simulink model "gtm_design"  (R2021b)
settings: Solver=VariableStepAuto  StartTime=0.0  StopTime=30  MinStep=0.0049  RelTol=1e-3
StopFcn:
  | MWSout=grabmws(bdroot);
  | MWSout.lastrun=datestr(now);
values from neighbouring files (symbols this model uses):
  g = 32.17405    [SingleDOF.m]    (also in layer1atm.m; mainSimple.m = 32.174; simio.m = [dx(Index.EOM(1:6)); delta(:)-f; -delta(:)-f ])
  GuidanceMode = 1    [mainSimple.m]    (also in setup.m)
  knots2fps = 1/fps2knots    (= 1.687800745)    [main.m]    (also in mainSimple.m = 1.68781)
  s = tf('s')    [SingleDOF.m]    (also in main.m; mainSimple.m; newmain.m)
undefined symbols (not defined in the file or in its folder): Aero, aftfuel, aftfuel_pos, AILL, AILLC, AILR, AILRC, alpha_deg, altitude_ft, Ax_g, Ay_g, Az_g, b, beta_deg, bias, BRAKEC, Cbar, cg_pos0, cg_shift_gear, DamageCase, DamageModels, DamageOnsetTime, Earth, ELLIB, ELLIBC, ELLOB, ELLOBC, ELRIB, ELRIBC, ELROB, ELROBC, engl_ang, engl_pos, engr_ang, engr_pos, FLAPLC, FLAPLIB, FLAPLOB, FLAPRC, FLAPRIB, FLAPROB, FuelUsed_Init, fwdfuel, fwdfuel_pos, GEAR, GEARC, Inertia0, Inertia_shift_gear, Ixx_model, Iyy_model, Izz_model, KTAS, LandingGear, LengON, LinearizeModeOn, m, MORPHLC, MORPHRC, NAV_altitude_m, NAV_latitude_deg ... (+51)
libraries: simulink_extras x39, simulink_need_slupdate x30, LPVBlockLibrary x9, aerolibconvert2 x7, simulink x3, aerolibtransform2 x3, UserContent_lib x2, uavalgslib x2, robotcorelib x1, uavutilslib x1
(part 1 of 7)
settings Model: VariantFading=off  LastModifiedBy=Jihoon Lee
settings DataIOCC: ReturnWorkspaceOutputs=off
settings OptimizationCC: BlockReduction=off  BooleanDataType=off
settings DebuggingCC: SaveWithParameterizedLinksMsg=none  UnderspecifiedInitializationDetection=Classic  MergeDetectMultiDrivingBlocksExec=none  SignalResolutionControl=TryResolveAllWithWarning
settings HardwareCC: TargetUnknown=on
settings ModelReferenceCC: PropagateSignalLabelsOutOfModel=off

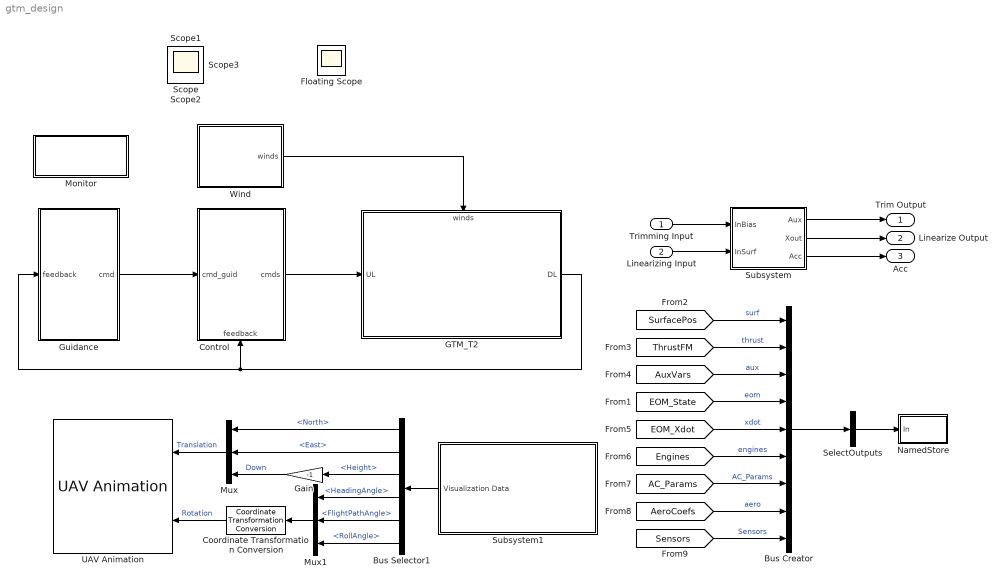
== system gtm_design ==
  Trimming Input : Inport  OutDataTypeStr=double  PortDimensions=4
  Linearizing Input : Inport  Port=2  OutDataTypeStr=double  PortDimensions=19
  Bus Creator : BusCreator  Inputs=9
  Bus Selector1 : BusSelector  OutputSignals=North,East,Height,HeadingAngle,FlightPathAngle,RollAngle
  Control : Subsystem
      settings: PortSchema="{\"entries\":[{\"content\":{\"sides\":[{\"content\":{\"connectorIds\":[\"In1\"]},\"type\":\"ConnectorPlacement.EquallySpacedRectSide\",\"uuid\":\"876f9d1c-31d1-4d48-8cbb-f6088518770e\"},{\"content\":{\"connectorIds\":[\"Out1\"],\"side\":\"RIGHT\"},\"type\":\"ConnectorPlacement.EquallySpacedRectSide\",\"uuid\":\"0e4266e3-a031-465f-8381-066e8420e2a4\"},{\"content\":{\"connectorIds\":[],\"side\":\"TOP\"},\"type\":\"ConnectorPlacement.EquallySpacedRectSide\",\"uuid\":\"3957ab9c-ff96-432b-bd6f-14b7cf2f8092\"},{\"content\":{\"connectorIds\":[\"In2\"],\"side\":\"BOTTOM\"},\"type\":\"ConnectorPlacement.EquallySpacedRectSide\",\"uuid\":\"1e447cfa-7c82-4ae0-9a3c-28fe1a02d81e\"}]},\"type\":\"ConnectorPlacement.EquallySpacedConnector\",\"uuid\":\"5c345d19-69a3-46c5-b9cf-f35f763eae5c\"}],\"packageUris\":[\"http://schema.mathworks.com/mf0/Connector/R2020b\"],\"version\":\"1.0\"}"
  Coordinate Transformation Conversion : robotcorelib/Coordinate Transformation Conversion  InputRepresentation=Euler Angles  InputEulerSequence=ZYX  ShowTrVecInputPort=on  OutputRepresentation=Quaternion  OutputEulerSequence=ZYX  ShowTrVecOutputPort=on  SimulateUsing=Code generation
      settings: SourceProductBaseCode=NV,RO,RR,UV
  GTM_T2 : Subsystem  Tag=From trunk/GTMsim/gtm_model.mdl revision 162
      settings: PortSchema="{\"entries\":[{\"content\":{\"sides\":[{\"content\":{\"connectorIds\":[\"In1\"]},\"type\":\"ConnectorPlacement.EquallySpacedRectSide\",\"uuid\":\"38bba5f1-4a0f-4ecd-874d-3a7e9850121a\"},{\"content\":{\"connectorIds\":[\"Out1\"],\"side\":\"RIGHT\"},\"type\":\"ConnectorPlacement.EquallySpacedRectSide\",\"uuid\":\"3320f707-8849-454c-b6a8-a1a5600dce96\"},{\"content\":{\"connectorIds\":[\"In2\"],\"side\":\"TOP\"},\"type\":\"ConnectorPlacement.EquallySpacedRectSide\",\"uuid\":\"e35b4c5d-b5fc-496b-a614-8f47a0366b54\"}]},\"type\":\"ConnectorPlacement.EquallySpacedConnector\",\"uuid\":\"76f2ccd8-2b0a-475c-a3e4-032abf049833\"}],\"packageUris\":[\"http://schema.mathworks.com/mf0/Connector/R2020b\"],\"version\":\"1.0\"}"
      mask Display: image(imread('GTMtiny.png'))
  Gain : Gain  Gain=-1
  Guidance : Subsystem
  Monitor : Subsystem
  Mux : Mux  Inputs=3
  Mux1 : Mux  Inputs=3
  NamedStore : Subsystem  StopFcn=|  mask{enable_logging=on, do_stopfcn_callback=on}
      | % if strmatch(get_param(gcb,'do_stopfcn_callback'),...
      | % 'on','exact')                                       
      | %    if exist('logsout','var')                        
      | %        sout = CreateSimOut(logsout);                
      | %    else                                             
      | %         %disp('No Log Data Variable')               
      | %     end                                             
      | % clear logsout                                       
      | % end
      mask prompts: enable_logging "Enable Data Logging"; do_stopfcn_callback "Post-process logsout"
      mask help: Produces signal log of input data. If post processing is selected the logsout object is converted into a data structure (sout) with fields named after the bus signals. In this case a common time base is recommended.
      mask init:
      | H=get_param([gcb,'/In'],'PortHandles');
      | if (enable_logging)
      |     set(H.Outport(1),'DataLogging','on')
      | else
      |     set(H.Outport(1),'DataLogging','off')
      |     
      | end
  SelectOutputs : BusSelector  OutputSignals=surf,thrust,aux,eom,xdot,engines,AC_Params,aero,Sensors  OutputAsBus=on
  Subsystem : Subsystem
  Subsystem1 : Subsystem
  UAV Animation : uavutilslib/UAV Animation  UAVType=FixedWing  UAVSize=50  InertialZDirection=Down  SampleTime=1
      settings: SourceProductBaseCode=UV
  Wind : Subsystem
  Trim Output : Outport  OutDataTypeStr=double  PortDimensions=6
  Linearize Output : Outport  Port=2  OutDataTypeStr=double  PortDimensions=12
  Acc : Outport  Port=3  OutDataTypeStr=double  PortDimensions=3
  Floating Scope : Scope
  Scope{,1..3} (4 alike) : Scope
  wires:
  Linearizing Input/1 -> Subsystem/2(InSurf)
  Subsystem/1(Aux) -> Trim Output/1
  Subsystem/2(Xout) -> Linearize Output/1
  Trimming Input/1 -> Subsystem/1(InBias)
  Control/1(cmds) -> GTM_T2/1(UL)
  Subsystem/3(Acc) -> Acc/1
  Bus Selector1/6 -> Mux1/3  "<RollAngle>"
  Mux/1 -> UAV Animation/1  "Translation"
  Bus Selector1/2 -> Mux/2  "<East>"
  Mux1/1 -> Coordinate Transformation Conversion/1
  Bus Selector1/1 -> Mux/1  "<North>"
  Bus Selector1/4 -> Mux1/1  "<HeadingAngle>"
  Coordinate Transformation Conversion/1 -> UAV Animation/2  "Rotation"
  Bus Selector1/3 -> Gain/1  "<Height>"
  Bus Selector1/5 -> Mux1/2  "<FlightPathAngle>"
  Gain/1 -> Mux/3  "Down"
  GTM_T2/1(DL) -> Guidance/1(feedback), Control/2(feedback)
  Guidance/1(cmd) -> Control/1(cmd_guid)
  Subsystem1/1(Visualization Data) -> Bus Selector1/1
  SelectOutputs/1 -> NamedStore/1(In)
  [AuxVars] -> Bus Creator/3  "aux"
  [ThrustFM] -> Bus Creator/2  "thrust"
  Bus Creator/1 -> SelectOutputs/1
  [SurfacePos] -> Bus Creator/1  "surf"
  [Sensors] -> Bus Creator/9  "Sensors"
  [Engines] -> Bus Creator/6  "engines"
  [EOM_Xdot] -> Bus Creator/5  "xdot"
  [AeroCoefs] -> Bus Creator/8  "aero"
  [AC_Params] -> Bus Creator/7  "AC_Params"
  [EOM_State] -> Bus Creator/4  "eom"
  Wind/1(winds) -> GTM_T2/2(winds)

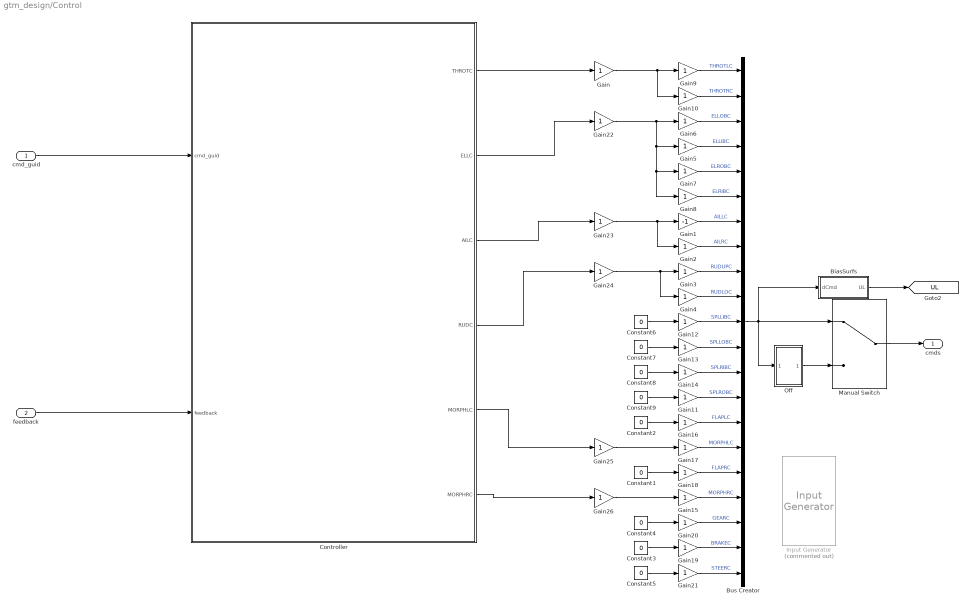
== system gtm_design/Control ==
  cmd_guid : Inport
  feedback : Inport  Port=2
  BiasSurfs : Subsystem
  Bus Creator : BusCreator  Inputs=21
  Constant{1..9} (9 alike) : Constant  Value=0
  Controller : Subsystem
  Gain{,22..26} (6 alike) : Gain
  Gain1 : Gain  Gain=-1  SaturateOnIntegerOverflow=on  OutDataTypeStr=Inherit: Same as input  ParamDataTypeStr=Inherit: Same as input
  Gain{2..21} (20 alike) : Gain  SaturateOnIntegerOverflow=on  OutDataTypeStr=Inherit: Same as input  ParamDataTypeStr=Inherit: Same as input
  Input Generator : UserContent_lib/Input Generator  Commented=on  SystemSampleTime=-1  VariantActivationTime=update diagram  Latency=0  AutoFrameSizeCalculation=off
      link override Doublet Generator: timeon=[2 12 7]  pulsewidth=[0.5 0.5 0.5]  amplitude=[0 0 0]
  Manual Switch : ManualSwitch
  Off : Subsystem
  cmds : Outport
  tag scope: UL=global
  wires:
  Gain9/1 -> Bus Creator/1  "THROTLC"
  Gain17/1 -> Bus Creator/16  "MORPHLC"
  Gain5/1 -> Bus Creator/4  "ELLIBC"
  Gain20/1 -> Bus Creator/19  "GEARC"
  Gain11/1 -> Bus Creator/14  "SPLROBC"
  Gain8/1 -> Bus Creator/6  "ELRIBC"
  Gain13/1 -> Bus Creator/12  "SPLLOBC"
  Gain1/1 -> Bus Creator/7  "AILLC"
  Gain7/1 -> Bus Creator/5  "ELROBC"
  Gain15/1 -> Bus Creator/18  "MORPHRC"
  Constant4/1 -> Gain20/1
  Gain2/1 -> Bus Creator/8  "AILRC"
  Gain3/1 -> Bus Creator/9  "RUDUPC"
  Gain21/1 -> Bus Creator/21  "STEERC"
  Gain14/1 -> Bus Creator/13  "SPLRIBC"
  Constant3/1 -> Gain19/1
  Gain6/1 -> Bus Creator/3  "ELLOBC"
  Gain10/1 -> Bus Creator/2  "THROTRC"
  Gain19/1 -> Bus Creator/20  "BRAKEC"
  Gain18/1 -> Bus Creator/17  "FLAPRC"
  Gain4/1 -> Bus Creator/10  "RUDLOC"
  Bus Creator/1 -> Off/1(In1), BiasSurfs/1(dCmd), Manual Switch/1
  Gain12/1 -> Bus Creator/11  "SPLLIBC"
  Gain16/1 -> Bus Creator/15  "FLAPLC"
  Constant2/1 -> Gain16/1
  Controller/3(AILC) -> Gain23/1
  Controller/2(ELLC) -> Gain22/1
  Controller/4(RUDC) -> Gain24/1
  Controller/1(THROTC) -> Gain/1
  cmd_guid/1 -> Controller/1(cmd_guid)
  feedback/1 -> Controller/2(feedback)
  Constant1/1 -> Gain18/1
  Constant5/1 -> Gain21/1
  Constant6/1 -> Gain12/1
  Constant7/1 -> Gain13/1
  Constant8/1 -> Gain14/1
  Constant9/1 -> Gain11/1
  Controller/5(MORPHLC) -> Gain25/1
  Controller/6(MORPHRC) -> Gain26/1
  Gain/1 -> Gain10/1, Gain9/1
  Gain22/1 -> Gain8/1, Gain7/1, Gain5/1, Gain6/1
  Gain23/1 -> Gain2/1, Gain1/1
  Gain24/1 -> Gain4/1, Gain3/1
  Gain25/1 -> Gain17/1
  Gain26/1 -> Gain15/1
  Manual Switch/1 -> cmds/1
  Off/1(Out1) -> Manual Switch/2
  BiasSurfs/1(UL) -> [UL]

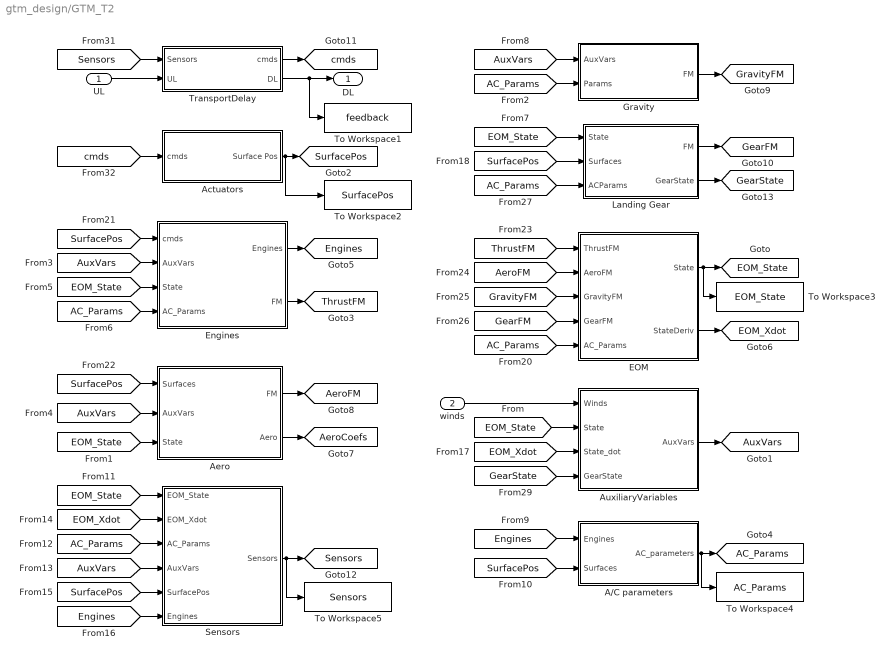
== system gtm_design/GTM_T2 ==
  UL : Inport
  winds : Inport  Port=2  PortDimensions=6
  A/C parameters : Subsystem
  Actuators : Subsystem
  Aero : Subsystem
  AuxiliaryVariables : Subsystem
  EOM : Subsystem
  Engines : Subsystem
  Gravity : Subsystem
  Landing Gear : Subsystem
  Sensors : Subsystem
  To Workspace1 : ToWorkspace  VariableName=feedback  SampleTime=-1
  To Workspace2 : ToWorkspace  VariableName=SurfacePos  SampleTime=-1
  To Workspace3 : ToWorkspace  VariableName=EOM_State  SampleTime=-1
  To Workspace4 : ToWorkspace  VariableName=AC_Params  SampleTime=-1
  To Workspace5 : ToWorkspace  VariableName=Sensors  SampleTime=-1
  TransportDelay : Subsystem
  DL : Outport
  tag scope: AC_Params=global, AeroCoefs=global, AeroFM=global, AuxVars=global, EOM_State=global, EOM_Xdot=global, Engines=global, GearFM=global, GearState=global, GravityFM=global, Sensors=global, SurfacePos=global, ThrustFM=global, cmds=global
  wires:
  UL/1 -> TransportDelay/2(UL)
  TransportDelay/2(DL) -> To Workspace1/1, DL/1
  Gravity/1(FM) -> [GravityFM]
  [AuxVars] -> Sensors/4(AuxVars)
  [EOM_Xdot] -> Sensors/2(EOM_Xdot)
  [Engines] -> Sensors/6(Engines)
  [SurfacePos] -> Sensors/5(SurfacePos)
  [AC_Params] -> Sensors/3(AC_Params)
  [EOM_State] -> Sensors/1(EOM_State)
  [AC_Params] -> EOM/5(AC_Params)
  [GearFM] -> EOM/4(GearFM)
  [GravityFM] -> EOM/3(GravityFM)
  [AeroFM] -> EOM/2(AeroFM)
  [ThrustFM] -> EOM/1(ThrustFM)
  [EOM_State] -> AuxiliaryVariables/2(State)
  [SurfacePos] -> Aero/1(Surfaces)
  [AC_Params] -> Landing Gear/3(ACParams)
  [SurfacePos] -> Engines/1(cmds)
  EOM/2(StateDeriv) -> [EOM_Xdot]
  [EOM_Xdot] -> AuxiliaryVariables/3(State_dot)
  Engines/1(Engines) -> [Engines]
  [SurfacePos] -> A/C parameters/2(Surfaces)
  [Engines] -> A/C parameters/1(Engines)
  A/C parameters/1(AC_parameters) -> To Workspace4/1, [AC_Params]
  [AC_Params] -> Engines/4(AC_Params)
  [AuxVars] -> Engines/2(AuxVars)
  [EOM_State] -> Engines/3(State)
  [AuxVars] -> Gravity/1(AuxVars)
  [AC_Params] -> Gravity/2(Params)
  EOM/1(State) -> To Workspace3/1, [EOM_State]
  Engines/2(FM) -> [ThrustFM]
  Aero/1(FM) -> [AeroFM]
  [AuxVars] -> Aero/2(AuxVars)
  AuxiliaryVariables/1(AuxVars) -> [AuxVars]
  [EOM_State] -> Aero/3(State)
  [EOM_State] -> Landing Gear/1(State)
  [SurfacePos] -> Landing Gear/2(Surfaces)
  Landing Gear/1(FM) -> [GearFM]
  Actuators/1(Surface Pos) -> To Workspace2/1, [SurfacePos]
  winds/1 -> AuxiliaryVariables/1(Winds)
  TransportDelay/1(cmds) -> [cmds]
  [Sensors] -> TransportDelay/1(Sensors)
  [cmds] -> Actuators/1(cmds)
  Sensors/1(Sensors) -> To Workspace5/1, [Sensors]
  Landing Gear/2(GearState) -> [GearState]
  [GearState] -> AuxiliaryVariables/4(GearState)
  Aero/2(Aero) -> [AeroCoefs]

== system gtm_design/Guidance ==
  feedback : Inport
  Airspeed Step : Subsystem  TreatAsAtomicUnit=on
  Elevation Step : Subsystem  TreatAsAtomicUnit=on
  GuidanceMode : Constant  Value=GuidanceMode
  "Invalid, Error Out" : Subsystem  TreatAsAtomicUnit=on
  Label : Subsystem
  Level Flight : Subsystem  TreatAsAtomicUnit=on
  Merge : Merge  Inputs=7
  Merge1 : Merge  InitialOutput=zeros(3,1)
  Merge2 : Merge  InitialOutput=zeros(1,1)
  Orbit Following : Subsystem  TreatAsAtomicUnit=on
  Roll Step : Subsystem  TreatAsAtomicUnit=on
  Switch Case : SwitchCase  CaseConditions={1,2,3,4,5,6}
  Terminator : Terminator
  Terminator1 : Terminator
  To Workspace : ToWorkspace  VariableName=command  SampleTime=-1
  Waypoint Following : Subsystem  TreatAsAtomicUnit=on
  cmd : Outport
  tag scope: DesiredCourse=global, GuidanceCmd=global, LookaheadPoint=global
  wires:
  Merge/1 -> Label/1(I)
  "Invalid, Error Out"/1(Out) -> Merge/7
  Waypoint Following/1(GuidanceCommand) -> Merge/5
  Roll Step/1(GuidanceCommand) -> Merge/4
  Airspeed Step/1(GuidanceCommand) -> Merge/3
  Elevation Step/1(GuidanceCommand) -> Merge/2
  Level Flight/1(GuidanceCommand) -> Merge/1
  Orbit Following/1(GuidanceCommand) -> Merge/6
  Switch Case/7 -> "Invalid, Error Out"/Action
  Switch Case/4 -> Roll Step/Action
  Switch Case/3 -> Airspeed Step/Action
  Switch Case/2 -> Elevation Step/Action
  Switch Case/6 -> Orbit Following/Action
  Switch Case/1 -> Level Flight/Action
  Switch Case/5 -> Waypoint Following/Action
  feedback/1 -> Orbit Following/1(Feedback), Waypoint Following/1(Feedback)
  GuidanceMode/1 -> Switch Case/1
  Merge2/1 -> [DesiredCourse]
  Merge1/1 -> [LookaheadPoint]
  Label/1(O) -> [GuidanceCmd], cmd/1, To Workspace/1
  Waypoint Following/2(LookaheadPoint) -> Merge1/1
  Orbit Following/2(LookaheadPoint) -> Merge1/2
  Orbit Following/3(DesiredCourse) -> Merge2/2
  Waypoint Following/3(DesiredCourse) -> Merge2/1
  [DesiredCourse] -> Terminator1/1
  [LookaheadPoint] -> Terminator/1

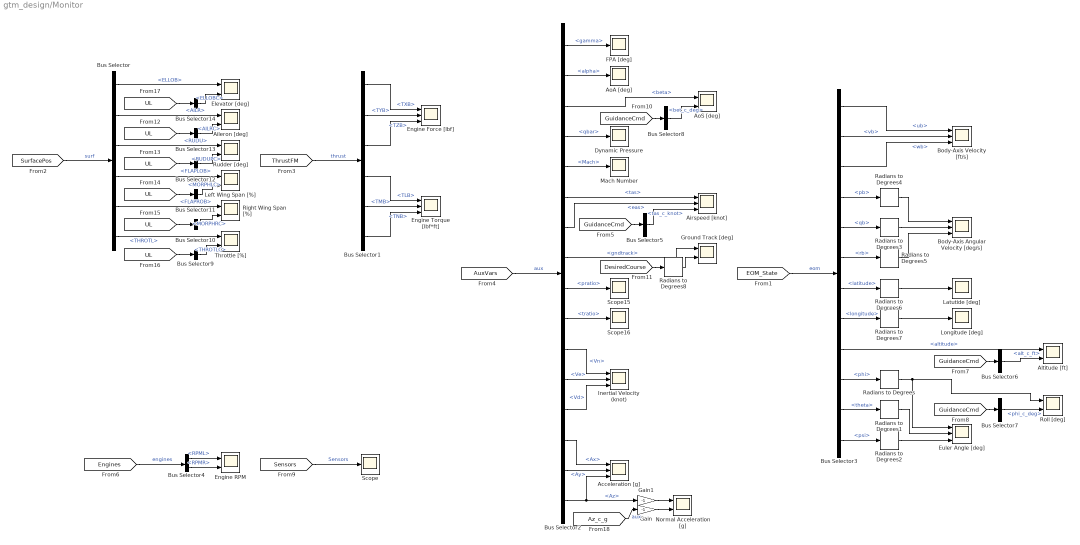
== system gtm_design/Monitor ==
  Acceleration [g] : Scope  NumInputPorts=3
  Aileron [deg] : Scope  NumInputPorts=2
  Airspeed [knot] : Scope  NumInputPorts=3
  Altitude [ft] : Scope  NumInputPorts=2
  AoA [deg] : Scope
  AoS [deg] : Scope  NumInputPorts=2
  Body-Axis Angular Velocity [deg/s] : Scope  NumInputPorts=3
  Body-Axis Velocity [ft/s] : Scope  NumInputPorts=3
  Bus Selector : BusSelector  OutputSignals=ELLOB,AILR,RUDU,FLAPLOB,FLAPROB,THROTL
  Bus Selector1 : BusSelector  OutputSignals=TXB,TYB,TZB,TLB,TMB,TNB
  Bus Selector10 : BusSelector  OutputSignals=MORPHRC
  Bus Selector11 : BusSelector  OutputSignals=MORPHLC
  Bus Selector12 : BusSelector  OutputSignals=RUDUPC
  Bus Selector13 : BusSelector  OutputSignals=AILRC
  Bus Selector14 : BusSelector  OutputSignals=ELLOBC
  Bus Selector2 : BusSelector  OutputSignals=gamma,alpha,beta,qbar,Mach,tas,eas,gndtrack,pratio,tratio,Vn,Ve,Vd,Ax,Ay,Az
  Bus Selector3 : BusSelector  OutputSignals=ub,vb,wb,pb,qb,rb,latitude,longitude,altitude,phi,theta,psi
  Bus Selector4 : BusSelector  OutputSignals=RPML,RPMR
  Bus Selector5 : BusSelector  OutputSignals=tas_c_knot
  Bus Selector6 : BusSelector  OutputSignals=alt_c_ft
  Bus Selector7 : BusSelector  OutputSignals=phi_c_deg
  Bus Selector8 : BusSelector  OutputSignals=bet_c_deg
  Bus Selector9 : BusSelector  OutputSignals=THROTLC
  Dynamic Pressure : Scope
  Elevator [deg] : Scope  NumInputPorts=2
  Engine Force [lbf] : Scope  NumInputPorts=3
  Engine RPM : Scope  NumInputPorts=2
  Engine Torque [lbf*ft] : Scope  NumInputPorts=3
  Euler Angle [deg] : Scope  NumInputPorts=3
  FPA [deg] : Scope
  Gain : Gain  Gain=-1
  Gain1 : Gain  Gain=-1
  Ground Track [deg] : Scope  NumInputPorts=2
  Inertial Velocity (knot) : Scope  NumInputPorts=3
  Latutide [deg] : Scope
  Left Wing Span [%] : Scope  NumInputPorts=2
  Longitude [deg] : Scope
  Mach Number : Scope
  Normal Acceleration [g] : Scope  NumInputPorts=2
  Radians to Degrees{,1..8} (9 alike) : simulink_extras/Transformations/Radians to Degrees
  Right Wing Span [%] : Scope  NumInputPorts=2
  Roll [deg] : Scope  NumInputPorts=2
  Rudder [deg] : Scope  NumInputPorts=2
  Scope : Scope
  Scope15 : Scope
  Scope16 : Scope
  Throttle [%] : Scope  NumInputPorts=2
  wires:
  [EOM_State] -> Bus Selector3/1  "eom"
  [Engines] -> Bus Selector4/1  "engines"
  [SurfacePos] -> Bus Selector/1  "surf"
  [ThrustFM] -> Bus Selector1/1  "thrust"
  [AuxVars] -> Bus Selector2/1  "aux"
  [Sensors] -> Scope/1  "Sensors"
  Bus Selector/1 -> Elevator [deg]/1  "<ELLOB>"
  Bus Selector/2 -> Aileron [deg]/1  "<AILR>"
  Bus Selector/3 -> Rudder [deg]/1  "<RUDU>"
  Bus Selector/4 -> Left Wing Span [%]/1  "<FLAPLOB>"
  Bus Selector/5 -> Right Wing Span [%]/1  "<FLAPROB>"
  Bus Selector/6 -> Throttle [%]/1  "<THROTL>"
  Bus Selector1/2 -> Engine Force [lbf]/2  "<TYB>"
  Bus Selector1/5 -> Engine Torque [lbf*ft]/2  "<TMB>"
  Bus Selector1/1 -> Engine Force [lbf]/1  "<TXB>"
  Bus Selector1/3 -> Engine Force [lbf]/3  "<TZB>"
  Bus Selector1/4 -> Engine Torque [lbf*ft]/1  "<TLB>"
  Bus Selector1/6 -> Engine Torque [lbf*ft]/3  "<TNB>"
  Bus Selector2/1 -> FPA [deg]/1  "<gamma>"
  Bus Selector2/2 -> AoA [deg]/1  "<alpha>"
  Bus Selector2/3 -> AoS [deg]/1  "<beta>"
  Bus Selector2/4 -> Dynamic Pressure/1  "<qbar>"
  Bus Selector2/5 -> Mach Number/1  "<Mach>"
  Bus Selector2/8 -> Ground Track [deg]/1  "<gndtrack>"
  Bus Selector2/9 -> Scope15/1  "<pratio>"
  Bus Selector2/10 -> Scope16/1  "<tratio>"
  Bus Selector2/12 -> Inertial Velocity (knot)/2  "<Ve>"
  Bus Selector2/14 -> Acceleration [g]/1  "<Ax>"
  Bus Selector2/6 -> Airspeed [knot]/1  "<tas>"
  Bus Selector2/7 -> Airspeed [knot]/2  "<eas>"
  Bus Selector2/15 -> Acceleration [g]/2  "<Ay>"
  Bus Selector2/11 -> Inertial Velocity (knot)/1  "<Vn>"
  Bus Selector2/13 -> Inertial Velocity (knot)/3  "<Vd>"
  Bus Selector2/16 -> Acceleration [g]/3, Gain1/1  "<Az>"
  Bus Selector3/8 -> Radians to Degrees7/1  "<longitude>"
  Bus Selector3/1 -> Body-Axis Velocity [ft/s]/1  "<ub>"
  Bus Selector3/9 -> Altitude [ft]/1  "<altitude>"
  Bus Selector3/2 -> Body-Axis Velocity [ft/s]/2  "<vb>"
  Bus Selector3/4 -> Radians to Degrees4/1  "<pb>"
  Bus Selector3/7 -> Radians to Degrees6/1  "<latitude>"
  Bus Selector3/3 -> Body-Axis Velocity [ft/s]/3  "<wb>"
  Bus Selector3/5 -> Radians to Degrees3/1  "<qb>"
  Bus Selector3/6 -> Radians to Degrees5/1  "<rb>"
  Bus Selector3/12 -> Radians to Degrees2/1  "<psi>"
  Bus Selector3/11 -> Radians to Degrees1/1  "<theta>"
  Bus Selector3/10 -> Radians to Degrees/1  "<phi>"
  Bus Selector4/1 -> Engine RPM/1  "<RPML>"
  Bus Selector4/2 -> Engine RPM/2  "<RPMR>"
  Radians to Degrees6/1 -> Latutide [deg]/1
  Radians to Degrees3/1 -> Body-Axis Angular Velocity [deg/s]/2
  Radians to Degrees4/1 -> Body-Axis Angular Velocity [deg/s]/1
  Radians to Degrees5/1 -> Body-Axis Angular Velocity [deg/s]/3
  Radians to Degrees7/1 -> Longitude [deg]/1
  Radians to Degrees/1 -> Euler Angle [deg]/1, Roll [deg]/1
  Radians to Degrees1/1 -> Euler Angle [deg]/2
  Radians to Degrees2/1 -> Euler Angle [deg]/3
  [GuidanceCmd] -> Bus Selector5/1
  Bus Selector5/1 -> Airspeed [knot]/3  "<tas_c_knot>"
  [GuidanceCmd] -> Bus Selector6/1
  Bus Selector6/1 -> Altitude [ft]/2  "<alt_c_ft>"
  [GuidanceCmd] -> Bus Selector7/1
  Bus Selector7/1 -> Roll [deg]/2  "<phi_c_deg>"
  [GuidanceCmd] -> Bus Selector8/1
  Bus Selector8/1 -> AoS [deg]/2  "<bet_c_deg>"
  [DesiredCourse] -> Radians to Degrees8/1
  Radians to Degrees8/1 -> Ground Track [deg]/2
  [UL] -> Bus Selector9/1
  Bus Selector9/1 -> Throttle [%]/2  "<THROTLC>"
  [UL] -> Bus Selector10/1
  [UL] -> Bus Selector11/1
  [UL] -> Bus Selector12/1
  [UL] -> Bus Selector13/1
  [UL] -> Bus Selector14/1
  Bus Selector14/1 -> Elevator [deg]/2  "<ELLOBC>"
  Bus Selector13/1 -> Aileron [deg]/2  "<AILRC>"
  Bus Selector12/1 -> Rudder [deg]/2  "<RUDUPC>"
  Bus Selector11/1 -> Left Wing Span [%]/2  "<MORPHLC>"
  Bus Selector10/1 -> Right Wing Span [%]/2  "<MORPHRC>"
  Gain1/1 -> Normal Acceleration [g]/1
  Gain/1 -> Normal Acceleration [g]/2
  [Az_c_g] -> Gain/1  "aux"

== system gtm_design/NamedStore ==
  In : Inport
  Terminator : Terminator
  wires:
  In/1 -> Terminator/1  "SimOut"

== system gtm_design/Subsystem ==
  InBias : Inport
  InSurf : Inport  Port=2
  Bus Selector : BusSelector  OutputSignals=eas,tas,alpha,beta,gamma,gndtrack  OutputAsBus=on
  Bus Selector1 : BusSelector  OutputSignals=Ax,Ay,Az  OutputAsBus=on
  Bus to Vector : BusToVector
  Bus to Vector1 : BusToVector
  Bus to Vector2 : BusToVector
  DocBlock : simulink/Model-Wide Utilities/DocBlock  DocumentType=Text
      content=|
      | Inputs and Outputs selected here have a specific ordering.
      |
      |
      |
      | Do not change this without also changing output channel ordering in associated linmodel.m and
      | trimgtm.m functions
  Aux : Outport
  Xout : Outport  Port=2
  Acc : Outport  Port=3
  tag scope: SurfaceBias=global, SurfaceDeltas=global
  wires:
  [EOM_State] -> Bus to Vector1/1  "eom"
  Bus Selector/1 -> Bus to Vector/1
  InSurf/1 -> [SurfaceDeltas]
  Bus to Vector/1 -> Aux/1
  Bus to Vector1/1 -> Xout/1
  InBias/1 -> [SurfaceBias]
  Bus to Vector2/1 -> Acc/1
  Bus Selector1/1 -> Bus to Vector2/1
  [AuxVars] -> Bus Selector1/1, Bus Selector/1  "aux"

== system gtm_design/Subsystem1 ==
  Bus Creator1 : BusCreator  Inputs=6
  Bus Selector1 : BusSelector  OutputSignals=latitude,longitude,altitude
  Bus Selector2 : BusSelector  OutputSignals=gndtrack,gamma
  Bus Selector3 : BusSelector  OutputSignals=phi
  Constant1 : Constant  Value=[37.827926944;-75.494061666]
  Constant2 : Constant  Value=0
  Constant3 : Constant  Value=0
  Degrees to Radians1 : simulink_extras/Transformations/Degrees to Radians
  Degrees to Radians2 : simulink_extras/Transformations/Degrees to Radians
  Demux1 : Demux  Outputs=3
      settings: DisplayOption=none
  Demux3 : Demux  Outputs=3
      settings: DisplayOption=none
  Gain : Gain  Gain=-1
  LLA to Flat Earth : aerolibtransform2/LLA to Flat Earth  units=English  ptype=Earth (WGS84)  F=1/298.257223563  R=20925646.3255  refPosPort=on  LL0=[0 10]  psi=0
      settings: SourceProductBaseCode=AE
  Mux : Mux  Inputs=3
  Mux2 : Mux  Inputs=2
  Radians to Degrees2 : simulink_extras/Transformations/Radians to Degrees
  To Workspace : ToWorkspace  VariableName=NED  SampleTime=-1
  Visualization Data : Outport
  wires:
  Demux1/3 -> Gain/1  "Down"
  Demux3/3 -> Bus Creator1/6  "RollAngle"
  Demux1/2 -> Bus Creator1/2  "East"
  Demux3/1 -> Bus Creator1/4  "HeadingAngle"
  Demux1/1 -> Bus Creator1/1  "North"
  Demux3/2 -> Bus Creator1/5  "FlightPathAngle"
  Bus Creator1/1 -> Visualization Data/1
  [EOM_State] -> Bus Selector1/1
  Gain/1 -> Bus Creator1/3  "Height"
  Bus Selector3/1 -> Mux/3  "<phi>"
  Degrees to Radians1/1 -> Mux/2  "gamma_rad"
  Degrees to Radians2/1 -> Mux/1  "gndtrack_rad"
  Mux/1 -> Demux3/1
  Constant3/1 -> LLA to Flat Earth/3
  Constant1/1 -> LLA to Flat Earth/4
  Constant2/1 -> LLA to Flat Earth/5
  Mux2/1 -> Radians to Degrees2/1
  Bus Selector1/3 -> LLA to Flat Earth/2  "<altitude>"
  [EOM_State] -> Bus Selector3/1  "eom"
  [AuxVars] -> Bus Selector2/1  "aux"
  Bus Selector2/1 -> Degrees to Radians2/1  "<gndtrack>"
  Bus Selector2/2 -> Degrees to Radians1/1  "<gamma>"
  Bus Selector1/1 -> Mux2/1  "<latitude>"
  Bus Selector1/2 -> Mux2/2  "<longitude>"
  LLA to Flat Earth/1 -> To Workspace/1, Demux1/1
  Radians to Degrees2/1 -> LLA to Flat Earth/1

== system gtm_design/Wind ==
  Bus Selector1 : BusSelector  OutputSignals=tas
  Bus Selector2 : BusSelector  OutputSignals=altitude
  Winds : UserContent_lib/Input Generator/Winds  WindSpeed_knots=WindSpd  WindDirection_deg=WindDir  level=None
  winds : Outport
  wires:
  Winds/1 -> winds/1
  [AuxVars] -> Bus Selector1/1
  [EOM_State] -> Bus Selector2/1
  Bus Selector1/1 -> Winds/2  "<tas>"
  Bus Selector2/1 -> Winds/1  "<altitude>"

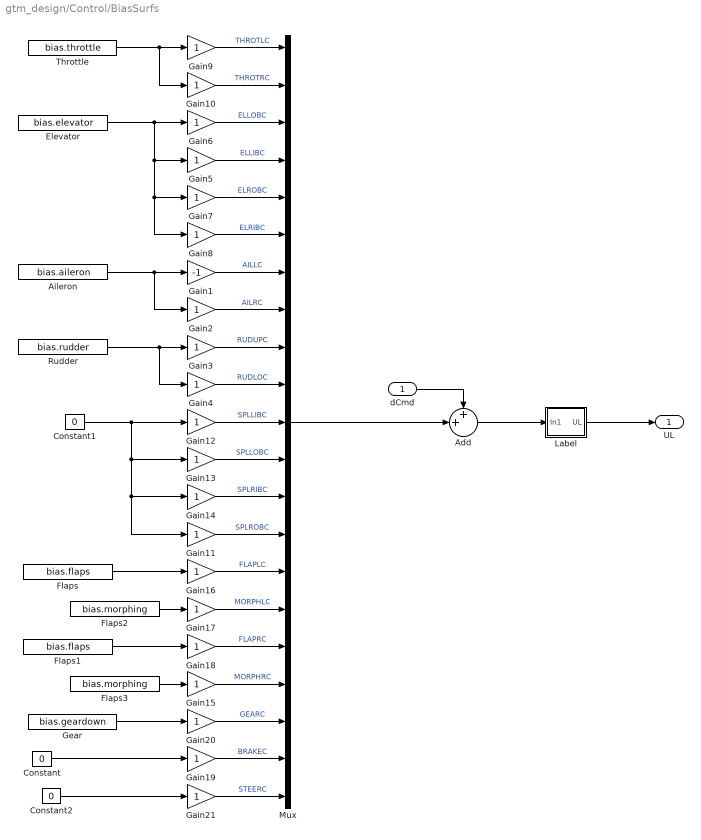
== system gtm_design/Control/BiasSurfs ==
  dCmd : Inport
  Add : Sum  Inputs=++|
  Aileron : Constant  Value=bias.aileron
  Constant : Constant  Value=0
  Constant1 : Constant  Value=0
  Constant2 : Constant  Value=0
  Elevator : Constant  Value=bias.elevator
  Flaps : Constant  Value=bias.flaps
  Flaps1 : Constant  Value=bias.flaps
  Flaps2 : Constant  Value=bias.morphing
  Flaps3 : Constant  Value=bias.morphing
  Gain1 : Gain  Gain=-1  SaturateOnIntegerOverflow=on  OutDataTypeStr=Inherit: Same as input  ParamDataTypeStr=Inherit: Same as input
  Gain{2..21} (20 alike) : Gain  SaturateOnIntegerOverflow=on  OutDataTypeStr=Inherit: Same as input  ParamDataTypeStr=Inherit: Same as input
  Gear : Constant  Value=bias.geardown
  Label : Subsystem
  Mux : Mux  Inputs=21
  Rudder : Constant  Value=bias.rudder
  Throttle : Constant  Value=bias.throttle
  UL : Outport
  wires:
  dCmd/1 -> Add/1
  Mux/1 -> Add/2
  Gain6/1 -> Mux/3  "ELLOBC"
  Flaps3/1 -> Gain15/1
  Gain7/1 -> Mux/5  "ELROBC"
  Flaps1/1 -> Gain18/1
  Gain18/1 -> Mux/17  "FLAPRC"
  Gain2/1 -> Mux/8  "AILRC"
  Constant1/1 -> Gain13/1, Gain11/1, Gain14/1, Gain12/1
  Gain11/1 -> Mux/14  "SPLROBC"
  Gain5/1 -> Mux/4  "ELLIBC"
  Gain8/1 -> Mux/6  "ELRIBC"
  Flaps2/1 -> Gain17/1
  Flaps/1 -> Gain16/1
  Rudder/1 -> Gain4/1, Gain3/1
  Gain14/1 -> Mux/13  "SPLRIBC"
  Gain17/1 -> Mux/16  "MORPHLC"
  Gain15/1 -> Mux/18  "MORPHRC"
  Gain4/1 -> Mux/10  "RUDLOC"
  Gain13/1 -> Mux/12  "SPLLOBC"
  Elevator/1 -> Gain8/1, Gain7/1, Gain5/1, Gain6/1
  Gain21/1 -> Mux/21  "STEERC"
  Gain19/1 -> Mux/20  "BRAKEC"
  Gain20/1 -> Mux/19  "GEARC"
  Gain3/1 -> Mux/9  "RUDUPC"
  Constant2/1 -> Gain21/1
  Throttle/1 -> Gain10/1, Gain9/1
  Gain12/1 -> Mux/11  "SPLLIBC"
  Constant/1 -> Gain19/1
  Gain16/1 -> Mux/15  "FLAPLC"
  Gear/1 -> Gain20/1
  Aileron/1 -> Gain2/1, Gain1/1
  Gain10/1 -> Mux/2  "THROTRC"
  Gain1/1 -> Mux/7  "AILLC"
  Gain9/1 -> Mux/1  "THROTLC"
  Add/1 -> Label/1(In1)
  Label/1(UL) -> UL/1

== system gtm_design/Control/Controller ==
  cmd_guid : Inport
  feedback : Inport  Port=2
  Bias Mixer : Subsystem
  Bus Selector : BusSelector  OutputSignals=tas_c_knot,alt_c_ft,bet_c_deg,phi_c_deg  OutputAsBus=on
  Bus Selector1 : BusSelector  OutputSignals=etas_c_percent  OutputAsBus=on
  Control Algorithm : Subsystem
  Demux : Demux  Outputs=6
  Morphing Mixer : Subsystem
  Mux : Mux  Inputs=6
  THROTC : Outport
  ELLC : Outport  Port=2
  AILC : Outport  Port=3
  RUDC : Outport  Port=4
  MORPHLC : Outport  Port=5
  MORPHRC : Outport  Port=6
  wires:
  cmd_guid/1 -> Bus Selector/1, Bus Selector1/1
  feedback/1 -> Control Algorithm/2(feedback)
  Control Algorithm/5(SPANAC) -> Morphing Mixer/1(SPANAC)
  Morphing Mixer/1(SPANLC) -> Mux/5
  Morphing Mixer/2(SPANRC) -> Mux/6
  Control Algorithm/3(AILC) -> Mux/3
  Control Algorithm/2(ELLC) -> Mux/2
  Control Algorithm/4(RUDC) -> Mux/4
  Control Algorithm/1(THROTC) -> Mux/1
  Mux/1 -> Bias Mixer/1(In)
  Bias Mixer/1(Out) -> Demux/1
  Demux/3 -> AILC/1
  Demux/4 -> RUDC/1
  Demux/2 -> ELLC/1
  Demux/5 -> MORPHLC/1
  Demux/1 -> THROTC/1
  Demux/6 -> MORPHRC/1
  Bus Selector/1 -> Control Algorithm/1(cmd_guid)
  Bus Selector1/1 -> Morphing Mixer/2(SPANSC)

== system gtm_design/Control/Off ==
  In1 : Inport
  Bus Creator : BusCreator  Inputs=21
  Demux : Demux  Outputs=21
  Gain27 : Gain  Gain=0
  Out1 : Outport
  wires:
  In1/1 -> Gain27/1
  Gain27/1 -> Demux/1
  Demux/11 -> Bus Creator/11  "SPLLIBC"
  Demux/21 -> Bus Creator/21  "STEERC"
  Demux/18 -> Bus Creator/18  "MORPHRC"
  Demux/15 -> Bus Creator/15  "FLAPLC"
  Demux/20 -> Bus Creator/20  "BRAKEC"
  Demux/10 -> Bus Creator/10  "RUDLOC"
  Demux/14 -> Bus Creator/14  "SPLROBC"
  Demux/13 -> Bus Creator/13  "SPLRIBC"
  Demux/5 -> Bus Creator/5  "ELROBC"
  Demux/12 -> Bus Creator/12  "SPLLOBC"
  Demux/2 -> Bus Creator/2  "THROTRC"
  Demux/4 -> Bus Creator/4  "ELLIBC"
  Demux/7 -> Bus Creator/7  "AILLC"
  Demux/19 -> Bus Creator/19  "GEARC"
  Demux/16 -> Bus Creator/16  "MORPHLC"
  Demux/3 -> Bus Creator/3  "ELLOBC"
  Demux/9 -> Bus Creator/9  "RUDUPC"
  Demux/17 -> Bus Creator/17  "FLAPRC"
  Demux/8 -> Bus Creator/8  "AILRC"
  Demux/1 -> Bus Creator/1  "THROTLC"
  Demux/6 -> Bus Creator/6  "ELRIBC"
  Bus Creator/1 -> Out1/1

== system gtm_design/GTM_T2/A//C parameters ==
  Engines : Inport
  Surfaces : Inport  Port=2
  B : Constant  Value=b
  Bus Creator4 : BusCreator  Inputs=15
  Bus Selector : BusSelector  OutputSignals=fuel_used
  Bus Selector1 : BusSelector  OutputSignals=GEAR
  Bus Selector2 : BusSelector  OutputSignals=SPLLOB,SPLROB  OutputAsBus=on
  Cbar : Constant  Value=Cbar
  Demux : Demux  Outputs=6
  Inertia/Mass/CG Shift : Subsystem  mask{DamageModels=DamageModels}
      mask prompts: DamageModels "Array of Damage Cases"
      mask init:
      | Ncases=length(DamageModels);
      | dCGDamage=zeros(Ncases+1,3);   
      | dMassDamage=zeros(Ncases+1,1);
      | dInertiaDamage=zeros(Ncases+1,6);
      | for i=1:Ncases,
      |   if isfield(DamageModels{i},'Mass'),
      |      dInertiaDamage(i+1,:)=DamageModels{i}.Mass.dIxxIyyIzzIxzIyzIxy;
      |      dCGDamage(i+1,:)=DamageModels{i}.Mass.dCG;
      |      dMassDamage(i+1)=DamageModels{i}.Mass.dWeight;
      |   end
      | end
  S : Constant  Value=S
  Surfaces1 : InportShadow  Port=2
  TriggerDamage : Subsystem
  ixxb5 : Constant  Value=engr_pos
  ixxb6 : Constant  Value=engl_pos
  xCG1 : Constant  Value=ref_cg
  AC_parameters : Outport
  wires:
  Bus Selector/1 -> Inertia/Mass/CG Shift/2(fuel_used)  "<fuel_used>"
  Bus Selector1/1 -> Inertia/Mass/CG Shift/1(gear)  "<GEAR>"
  [DamageCase] -> Inertia/Mass/CG Shift/3(DamageCase)
  [DamageCase] -> Bus Creator4/13  "DamageCase"
  Inertia/Mass/CG Shift/3(CG) -> Bus Creator4/12  "CG"
  Inertia/Mass/CG Shift/2(mass) -> Bus Creator4/11  "mass"
  Demux/6 -> Bus Creator4/10  "Ixy"
  Demux/5 -> Bus Creator4/9  "Iyz"
  Demux/4 -> Bus Creator4/8  "Ixz"
  Demux/3 -> Bus Creator4/7  "Izz"
  Demux/2 -> Bus Creator4/6  "Iyy"
  Demux/1 -> Bus Creator4/5  "Ixx"
  ixxb6/1 -> Bus Creator4/15  "LfEng"
  ixxb5/1 -> Bus Creator4/14  "RtEng"
  xCG1/1 -> Bus Creator4/4  "CP"
  B/1 -> Bus Creator4/3  "B"
  Cbar/1 -> Bus Creator4/2  "Cbar"
  S/1 -> Bus Creator4/1  "S"
  TriggerDamage/1(damagecase) -> [DamageCase]
  Inertia/Mass/CG Shift/1(Inertia) -> Demux/1
  Surfaces/1 -> Bus Selector1/1
  Engines/1 -> Bus Selector/1
  Bus Creator4/1 -> AC_parameters/1
  Surfaces1/1 -> Bus Selector2/1
  Bus Selector2/1 -> Inertia/Mass/CG Shift/4(morphing)

== system gtm_design/GTM_T2/Actuators ==
  cmds : Inport
  Acutator Dynamics : Subsystem
  DeadBand : Subsystem
  InputModification for Trimming : Subsystem
  Label : Subsystem
  TimeDelay with IC feedthrough : Subsystem
  Surface Pos : Outport
  wires:
  TimeDelay with IC feedthrough/1(O) -> InputModification for Trimming/1(CmdVec)
  DeadBand/1(O) -> Surface Pos/1
  cmds/1 -> Acutator Dynamics/1(In)
  [SurfaceDeltas] -> InputModification for Trimming/3(SurfaceDeltas)
  Label/1(O) -> DeadBand/1(I)
  [SurfaceBias] -> InputModification for Trimming/2(SurfBias)
  InputModification for Trimming/1(CmdVecOut) -> Label/1(I)
  Acutator Dynamics/1(Out) -> TimeDelay with IC feedthrough/1(I)

== system gtm_design/GTM_T2/Aero ==
  Surfaces : Inport
  AuxVars : Inport  Port=2
  State : Inport  Port=3
  Basic Airframe : Subsystem
  Bus Selector1 : BusSelector  OutputSignals=CG,CP
  Bus Selector2 : BusSelector  OutputSignals=alpha,beta
  Bus Selector3 : BusSelector  OutputSignals=alpha  OutputAsBus=on
  Bus Selector4 : BusSelector  OutputSignals=beta  OutputAsBus=on
  Bus Selector6 : BusSelector  OutputSignals=tas
  Bus Selector7 : BusSelector  OutputSignals=qbar
  Bus Selector8 : BusSelector  OutputSignals=pb,qb,rb  OutputAsBus=on
  Bus to Vector5 : BusToVector
  Coefficent Evaluation : Subsystem  mask{b=b, cbar=Cbar, Sref=S}
      mask prompts: b "Reference Span (b)"; cbar "Reference Chord (cbar)"; Sref "Reference Area (Sref)"
      mask help:
      | Calulates the Force and Moments due to aerodynamic loads from vector of body axes aerodynamic coefficients:
      |    C6body = [Cx Cy Cz Cl Cm Cn].
      | Also requires dynamic pressure, cg/cp locations and reference lengths/area.
  Control Surfaces : Subsystem
  Dynamic Derviatives : Subsystem
  Label : Subsystem
  Stall Rolling Moment Asymmetry : Subsystem
  Sum8 : Sum  Inputs=++++  InputSameDT=on  SaturateOnIntegerOverflow=on  OutDataTypeStr=Inherit: Same as first input
  stall_cl_asym_enabled : Constant  Value=stall_cl_asym_enabled
  symmetry_on : Constant  Value=symmetric_aero_on
  FM : Outport
  Aero : Outport  Port=2
  wires:
  [AC_Params] -> Dynamic Derviatives/5(AC_Params)
  Bus to Vector5/1 -> Dynamic Derviatives/4(pqr)
  Bus Selector6/1 -> Dynamic Derviatives/3(TAS)  "<tas>"
  [AC_Params] -> Basic Airframe/4(AC_Params)
  Bus Selector8/1 -> Bus to Vector5/1  "pqr"
  Basic Airframe/1(C6) -> Sum8/1
  Control Surfaces/1(dC6) -> Sum8/2
  Dynamic Derviatives/1(dC6) -> Sum8/3
  State/1 -> Bus Selector8/1
  Bus Selector2/2 -> Basic Airframe/2(beta), Dynamic Derviatives/2(beta), Control Surfaces/2(beta)  "<beta>"
  Bus Selector2/1 -> Basic Airframe/1(alpha), Dynamic Derviatives/1(alpha), Control Surfaces/1(alpha)  "<alpha>"
  AuxVars/1 -> Bus Selector2/1, Bus Selector6/1, Bus Selector3/1, Bus Selector7/1, Bus Selector4/1
  Label/1(O) -> FM/1
  Bus Selector7/1 -> Coefficent Evaluation/2(qbar)  "<qbar>"
  Sum8/1 -> Aero/1, Coefficent Evaluation/1(C6 Body)
  Coefficent Evaluation/1(Forces) -> Label/1(If)
  Coefficent Evaluation/2(Moments) -> Label/2(Im)
  Bus Selector1/1 -> Coefficent Evaluation/3(Cg)  "<CG>"
  [AC_Params] -> Bus Selector1/1
  Bus Selector1/2 -> Coefficent Evaluation/4(Cp)  "<CP>"
  symmetry_on/1 -> Basic Airframe/3(symmetry_on)
  Surfaces/1 -> Control Surfaces/3(surfaces)
  stall_cl_asym_enabled/1 -> Stall Rolling Moment Asymmetry/3(stall_cl_asym_enabled)
  Stall Rolling Moment Asymmetry/1(dC6) -> Sum8/4
  Bus Selector3/1 -> Stall Rolling Moment Asymmetry/1(alpha)
  Bus Selector4/1 -> Stall Rolling Moment Asymmetry/2(beta)
  [AC_Params] -> Control Surfaces/4(AC_Params)

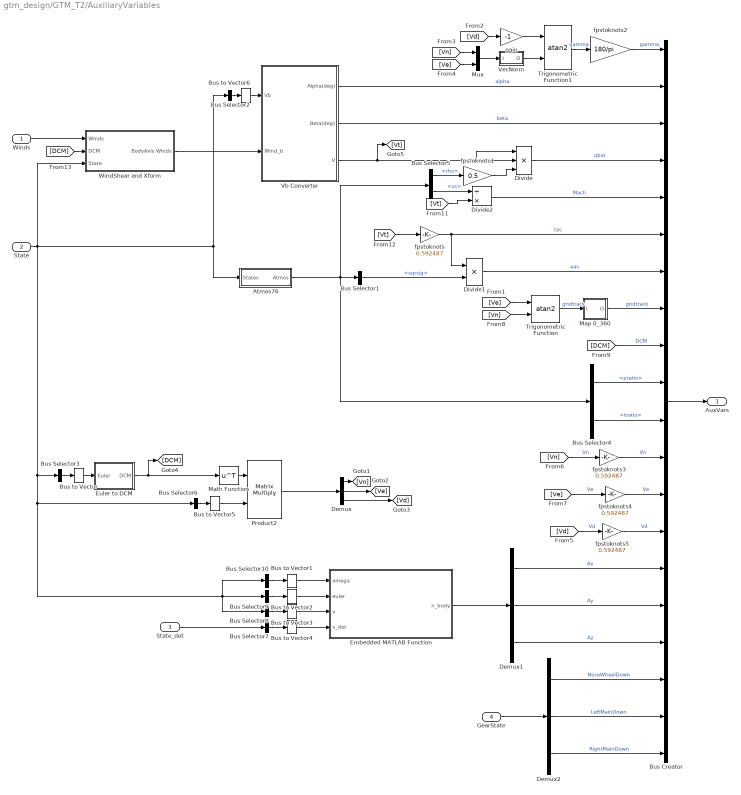
== system gtm_design/GTM_T2/AuxiliaryVariables ==
  Winds : Inport  PortDimensions=6
  State : Inport  Port=2
  State_dot : Inport  Port=3
  GearState : Inport  Port=4
  Atmos76 : Subsystem
  Bus Creator : BusCreator  Inputs=20
  Bus Selector1 : BusSelector  OutputSignals=sqrsig
  Bus Selector10 : BusSelector  OutputSignals=pb,qb,rb  OutputAsBus=on
  Bus Selector2 : BusSelector  OutputSignals=ub,vb,wb  OutputAsBus=on
  Bus Selector3 : BusSelector  OutputSignals=phi,theta,psi  OutputAsBus=on
  Bus Selector4 : BusSelector  OutputSignals=pratio,tratio
  Bus Selector5 : BusSelector  OutputSignals=rho,cs
  Bus Selector6 : BusSelector  OutputSignals=ub,vb,wb  OutputAsBus=on
  Bus Selector7 : BusSelector  OutputSignals=ub_dot,vb_dot,wb_dot  OutputAsBus=on
  Bus Selector8 : BusSelector  OutputSignals=ub,vb,wb  OutputAsBus=on
  Bus Selector9 : BusSelector  OutputSignals=phi,theta,psi  OutputAsBus=on
  Bus to Vector{,1..6} (7 alike) : BusToVector
  Demux : Demux  Outputs=3
  Demux1 : Demux  Outputs=3
  Demux2 : Demux  Outputs=3
  Divide : Product  Inputs=***
  Divide1 : Product
  Divide2 : Product  Inputs=/*
  Embedded MATLAB Function : MATLAB Function  TreatAsAtomicUnit=on
  Euler to DCM : Subsystem
  Map 0_360 : Subsystem
  Math Function : Math  Operator=transpose  SignedPower=on  SaturateOnIntegerOverflow=on
  Mux : Mux  Inputs=2
  Product2 : Product  Multiplication=Matrix(*)  RndMeth=Zero
  Trigonometric Function : Trigonometry  Operator=atan2
  Trigonometric Function1 : Trigonometry  Operator=atan2
  Vb Converter : Subsystem
  VecNorm : Subsystem
  WindShear and Xform : Subsystem
  fpstoknots{,3..5} (4 alike) : Gain  Gain=0.592487
  fpstoknots1 : Gain  Gain=0.5
  fpstoknots2 : Gain  Gain=180/pi
  gain : Gain  Gain=-1
  AuxVars : Outport
  wires:
  Demux2/3 -> Bus Creator/20  "RightMainDown"
  Demux2/2 -> Bus Creator/19  "LeftMainDown"
  Demux2/1 -> Bus Creator/18  "NoseWheelDown"
  GearState/1 -> Demux2/1
  [DCM] -> WindShear and Xform/2(DCM)
  WindShear and Xform/1(BodyAxis Winds) -> Vb Converter/2(Wind_b)
  Winds/1 -> WindShear and Xform/1(Winds)
  Product2/1 -> Demux/1
  Bus to Vector6/1 -> Vb Converter/1(Vb)
  Bus Selector2/1 -> Bus to Vector6/1
  Bus to Vector5/1 -> Product2/2
  Bus to Vector4/1 -> Embedded MATLAB Function/4(v_dot)
  Bus to Vector3/1 -> Embedded MATLAB Function/3(v)
  Bus to Vector2/1 -> Embedded MATLAB Function/2(euler)
  Bus to Vector1/1 -> Embedded MATLAB Function/1(omega)
  Bus to Vector/1 -> Euler to DCM/1("Euler ")
  Bus Selector3/1 -> Bus to Vector/1
  Bus Selector6/1 -> Bus to Vector5/1
  Math Function/1 -> Product2/1
  Demux/1 -> [Vn]
  Demux/2 -> [Ve]
  Embedded MATLAB Function/1(n_body) -> Demux1/1
  Demux1/3 -> Bus Creator/17  "Az"
  Demux1/2 -> Bus Creator/16  "Ay"
  Demux1/1 -> Bus Creator/15  "Ax"
  Bus Selector10/1 -> Bus to Vector1/1
  Bus Selector9/1 -> Bus to Vector2/1
  Bus Selector8/1 -> Bus to Vector3/1
  State_dot/1 -> Bus Selector7/1
  Bus Selector7/1 -> Bus to Vector4/1
  Bus Creator/1 -> AuxVars/1
  [Vt] -> fpstoknots/1
  [Vt] -> Divide2/2
  [DCM] -> Bus Creator/9  "DCM"
  fpstoknots5/1 -> Bus Creator/14  "Vd"
  fpstoknots4/1 -> Bus Creator/13  "Ve"
  fpstoknots3/1 -> Bus Creator/12  "Vn"
  Divide2/1 -> Bus Creator/5  "Mach"
  Bus Selector5/2 -> Divide2/1  "<cs>"
  Trigonometric Function/1 -> Map 0_360/1(I)  "gndtrack"
  Map 0_360/1(O) -> Bus Creator/8  "gndtrack"
  [Vn] -> Trigonometric Function/2
  [Ve] -> Trigonometric Function/1
  Bus Selector4/2 -> Bus Creator/11  "<tratio>"
  Bus Selector4/1 -> Bus Creator/10  "<pratio>"
  [Vd] -> fpstoknots5/1  "Vd"
  [Vn] -> fpstoknots3/1  "Vn"
  [Ve] -> fpstoknots4/1  "Ve"
  Divide1/1 -> Bus Creator/7  "eas"
  State/1 -> WindShear and Xform/3(State), Bus Selector3/1, Bus Selector6/1, Bus Selector8/1, Bus Selector10/1, Bus Selector9/1, Atmos76/1(States), Bus Selector2/1
  Atmos76/1(Atmos) -> Bus Selector4/1, Bus Selector1/1, Bus Selector5/1
  fpstoknots/1 -> Bus Creator/6, Divide1/1  "tas"
  Vb Converter/3(V) -> [Vt], Divide/1, Divide/2
  Bus Selector1/1 -> Divide1/2  "<sqrsig>"
  Vb Converter/1(Alpha(deg)) -> Bus Creator/2  "alpha"
  Vb Converter/2(Beta(deg)) -> Bus Creator/3  "beta"
  Bus Selector5/1 -> fpstoknots1/1  "<rho>"
  fpstoknots1/1 -> Divide/3
  Divide/1 -> Bus Creator/4  "qbar"
  Euler to DCM/1(DCM) -> Math Function/1, [DCM]
  Demux/3 -> [Vd]
  Trigonometric Function1/1 -> fpstoknots2/1  "gamma"
  gain/1 -> Trigonometric Function1/1
  [Vd] -> gain/1
  Mux/1 -> VecNorm/1(I)
  [Vn] -> Mux/1
  [Ve] -> Mux/2
  VecNorm/1(O) -> Trigonometric Function1/2
  fpstoknots2/1 -> Bus Creator/1  "gamma"

== system gtm_design/GTM_T2/EOM ==
  ThrustFM : Inport
  AeroFM : Inport  Port=2
  GravityFM : Inport  Port=3
  GearFM : Inport  Port=4
  AC_Params : Inport  Port=5
  Add : Sum  Inputs=++++
  Aircraft 6DOF : Subsystem  mask{UnitOfLength=ft}
      mask prompts: UnitOfLength "Length Unit"
      mask help:
      | Six Degree of Freedom Aircraft Simulation
      |
      | Input forces are both linear forces and torques -> [Fx Fy Fz Tl Tm Tn].
      | Inertia6 is a vector [Ixx Iyy Izz  Ixz Iyz Ixy], all positive
      | State Vector is [Vb pqr LatLonAlt PhiThetaPsi]
      mask init:
      | if (UnitOfLength==1), % ft
      |     Re=6.37043246e+06/.3048;
      | elseif (UnitOfLength==2), % m
      |     Re=6.37043246e+06;
      | end
      mask TypeOptions UnitOfLength: ft | meters
  Anti Windup : Subsystem
  Bus Selector1 : BusSelector  OutputSignals=Ixx,Iyy,Izz,Ixz,Iyz,Ixy  OutputAsBus=on
  Bus Selector11 : BusSelector  OutputSignals=mass
  Bus to Vector : BusToVector
  Bus to Vector1 : BusToVector
  Bus to Vector2 : BusToVector
  Integrator : Integrator  InitialCondition=StatesInp
  State Labels : Subsystem
  Xdot Labels : Subsystem
  State : Outport
  StateDeriv : Outport  Port=2
  wires:
  Bus to Vector2/1 -> Add/2
  Bus to Vector1/1 -> Add/1
  ThrustFM/1 -> Bus to Vector1/1
  AeroFM/1 -> Bus to Vector2/1
  State Labels/1(O) -> State/1
  Bus to Vector/1 -> Aircraft 6DOF/3(Inertia6)
  GearFM/1 -> Add/4
  GravityFM/1 -> Add/3
  Add/1 -> Aircraft 6DOF/1(Forces)
  Xdot Labels/1(O) -> StateDeriv/1
  Bus Selector1/1 -> Bus to Vector/1
  Aircraft 6DOF/1(Xdot) -> Xdot Labels/1(I), Integrator/1
  Anti Windup/1(O) -> State Labels/1(I)
  Integrator/1 -> Aircraft 6DOF/4(State), Anti Windup/1(I)
  Bus Selector11/1 -> Aircraft 6DOF/2(mass)  "<mass>"
  AC_Params/1 -> Bus Selector1/1, Bus Selector11/1

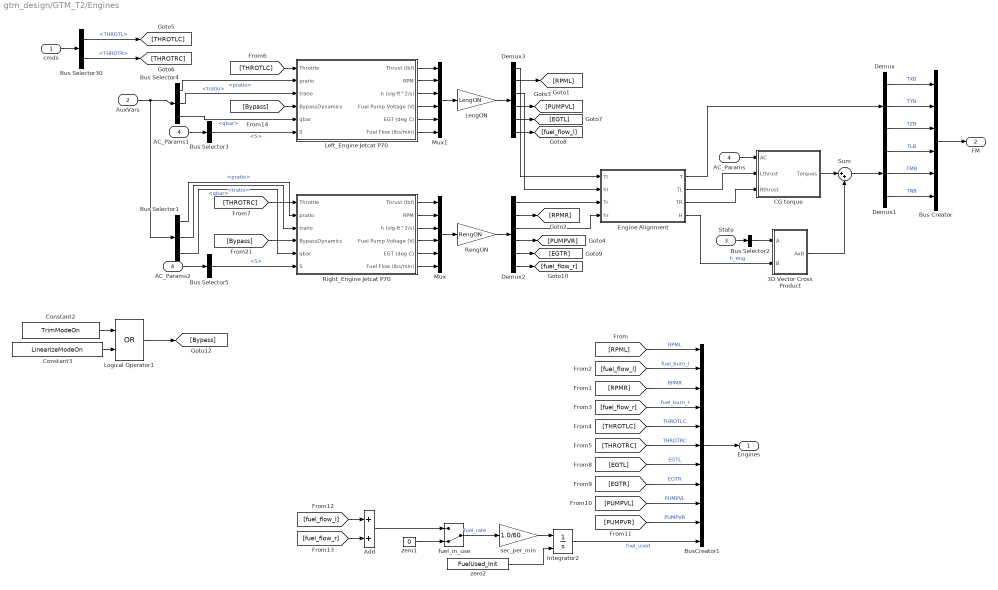
== system gtm_design/GTM_T2/Engines ==
  cmds : Inport
  AuxVars : Inport  Port=2
  State : Inport  Port=3
  AC_Params : Inport  Port=4
  3D Vector Cross Product : Subsystem
  AC_Params1 : InportShadow  Port=4
  AC_Params2 : InportShadow  Port=4
  Add : Sum
  Bus Creator : BusCreator  Inputs=6
  Bus Selector1 : BusSelector  OutputSignals=pratio,tratio,qbar
  Bus Selector2 : BusSelector  OutputSignals=pb,qb,rb  OutputAsBus=on
  Bus Selector3 : BusSelector  OutputSignals=S
  Bus Selector30 : BusSelector  OutputSignals=THROTL,THROTR
  Bus Selector4 : BusSelector  OutputSignals=pratio,tratio,qbar
  Bus Selector5 : BusSelector  OutputSignals=S
  BusCreator1 : BusCreator  Inputs=11
  CG torque : Subsystem
  Constant2 : Constant  Value=TrimModeOn
  Constant3 : Constant  Value=LinearizeModeOn
  Demux : Demux  Outputs=3
  Demux1 : Demux  Outputs=3
  Demux2 : Demux  Outputs=6
  Demux3 : Demux  Outputs=6
  Engine Alignment : MATLAB Function  TreatAsAtomicUnit=on
  Integrator2 : Integrator  InitialConditionSource=external
  Left_Engine Jetcat P70 : Subsystem
      mask init:
      | % Curve fit parameters for Jetcat P70 Model
      | % Coeff_thrust   = [0.000028864242464  -0.001914835880159 0.105916926095459  -1.251646340183624 ];
      | Coeff_thrust   = [0.000014847593013,  0, 0, 0.412662356277121];
      | Coeff_throttle = [0.000033035538475  -0.008354385314499 1.191126728328792 31.518959847101669];
      | Coeff_fuelflow = [0.000046800927870  -0.000779344124807 0.122178501497750];
      | Coeff_tau      = [ -2.2400e-02   2.9948e+00];
      | Coeff_EGT      = [ 2E-5, -0.0036,0.2342,-8.0496,664.99]; %EGT model, deg C
      | Coeff_dynamics = [ -.074 7.1];
      | fuelpump_table = [0 0.576	0.625	0.6985	0.7845	0.8575	0.919	0.9805	1.0415	1.1025...
      |                     1.1515	1.262	1.287	1.373	1.52	1.618	1.74	1.887	1.973...
      |                     2.12	2.255	2.4385	2.647	2.7575	2.9905	3.162]; %volts, table of fuel pump voltages
      | fuelflow_table = [0,0.0794,0.0876,0.102,0.1149,0.1275,0.1379,0.1487,0.1586,0.1671,...
      |                     0.1775,0.1858,0.194,0.2038,0.2206,0.2405,0.2566,0.2746,0.2921,0.3102,...
      |                     0.3266,0.3445,0.3533,0.3611,0.3866,0.4083;]*2; %lbs/min,   FULL fuel flow rates corresponding to pump voltages (fuelpump_table)  
      | % Equvalent Shaft parameters for engine
      | shaft_dia = 0.75/12.0;       % diameter of rotating turbine in feet 
      | shaft_len = 6.25/12.0;       % length of rotating turbine in feet   
      | density   = 15.2;            % mass density of steel in slugs/ft^3 
      | 
      | 
      | A = [-1.336,-0.7314;1,0;];
      | B = [1;0];
      | C = [-0.1474   0.7314];
      | D = 0;
  LengON : Gain  Gain=LengON  SaturateOnIntegerOverflow=on  OutDataTypeStr=Inherit: Same as input  ParamDataTypeStr=Inherit: Same as input
  Logical Operator1 : Logic  Operator=OR  AllPortsSameDT=off  OutDataTypeStr=boolean
  Mux : Mux  Inputs=6
  Mux1 : Mux  Inputs=6
  RengON : Gain  Gain=RengON  SaturateOnIntegerOverflow=on  OutDataTypeStr=Inherit: Same as input  ParamDataTypeStr=Inherit: Same as input
  Right_Engine Jetcat P70 : Subsystem
      mask init: same as gtm_design/GTM_T2/Engines/Left_Engine Jetcat P70
  Sum : Sum  Inputs=|++
  fuel_in_use : ManualSwitch  CurrentSetting=0
  sec_per_min : Gain  Gain=1.0/60.  SaturateOnIntegerOverflow=on  OutDataTypeStr=Inherit: Same as input  ParamDataTypeStr=Inherit: Same as input
  zero1 : Constant  Value=0
  zero2 : Constant  Value=FuelUsed_Init
  Engines : Outport
  FM : Outport  Port=2  PortDimensions=6
  wires:
  cmds/1 -> Bus Selector30/1
  Demux/2 -> Bus Creator/2  "TYB"
  State/1 -> Bus Selector2/1
  Bus Selector2/1 -> 3D Vector Cross Product/1(A)
  Demux/3 -> Bus Creator/3  "TZB"
  AuxVars/1 -> Bus Selector1/1, Bus Selector4/1
  AC_Params/1 -> CG torque/1(AC)
  Bus Creator/1 -> FM/1
  Bus Selector30/1 -> [THROTLC]  "<THROTL>"
  Bus Selector30/2 -> [THROTRC]  "<THROTR>"
  [THROTRC] -> BusCreator1/6  "THROTRC"
  [THROTLC] -> BusCreator1/5  "THROTLC"
  [fuel_flow_r] -> BusCreator1/4  "fuel_burn_r"
  [fuel_flow_l] -> BusCreator1/2  "fuel_burn_l"
  [RPMR] -> BusCreator1/3  "RPMR"
  [RPML] -> BusCreator1/1  "RPML"
  BusCreator1/1 -> Engines/1
  [EGTL] -> BusCreator1/7  "EGTL"
  [EGTR] -> BusCreator1/8  "EGTR"
  [PUMPVL] -> BusCreator1/9  "PUMPVL"
  [PUMPVR] -> BusCreator1/10  "PUMPVR"
  sec_per_min/1 -> Integrator2/1
  fuel_in_use/1 -> sec_per_min/1  "fuel_rate"
  Integrator2/1 -> BusCreator1/11  "fuel_used"
  zero2/1 -> Integrator2/2
  [fuel_flow_l] -> Add/1
  [fuel_flow_r] -> Add/2
  zero1/1 -> fuel_in_use/2
  Add/1 -> fuel_in_use/1
  Demux/1 -> Bus Creator/1  "TXB"
  Engine Alignment/4(H) -> 3D Vector Cross Product/2(B)  "h_eng"
  Engine Alignment/1(T) -> Demux/1
  Engine Alignment/2(TL) -> CG torque/2(Lthrust)
  Engine Alignment/3(TR) -> CG torque/3(Rthrust)
  CG torque/1(Torques) -> Sum/1
  3D Vector Cross Product/1(AxB) -> Sum/2
  Sum/1 -> Demux1/1
  Demux1/1 -> Bus Creator/4  "TLB"
  Demux1/2 -> Bus Creator/5  "TMB"
  Demux1/3 -> Bus Creator/6  "TNB"
  Mux/1 -> RengON/1
  RengON/1 -> Demux2/1
  Demux2/1 -> Engine Alignment/3(Tr)
  Demux2/2 -> [RPMR]
  Demux2/3 -> Engine Alignment/4(hr)
  Demux2/4 -> [PUMPVR]
  Demux2/5 -> [EGTR]
  Demux2/6 -> [fuel_flow_r]
  Mux1/1 -> LengON/1
  LengON/1 -> Demux3/1
  Demux3/1 -> Engine Alignment/1(Tl)
  Demux3/2 -> [RPML]
  Demux3/3 -> Engine Alignment/2(hl)
  Demux3/4 -> [PUMPVL]
  Demux3/5 -> [EGTL]
  Demux3/6 -> [fuel_flow_l]
  Constant3/1 -> Logical Operator1/2
  Constant2/1 -> Logical Operator1/1
  Logical Operator1/1 -> [Bypass]
  Left_Engine Jetcat P70/1(Thrust (lbf)) -> Mux1/1
  Left_Engine Jetcat P70/2(RPM) -> Mux1/2
  Left_Engine Jetcat P70/3(h (slg-ft^2/s)) -> Mux1/3
  Left_Engine Jetcat P70/4(Fuel Pump Voltage (V)) -> Mux1/4
  Left_Engine Jetcat P70/5(EGT (deg C)) -> Mux1/5
  Left_Engine Jetcat P70/6(Fuel Flow (lbs/min)) -> Mux1/6
  Right_Engine Jetcat P70/1(Thrust (lbf)) -> Mux/1
  Right_Engine Jetcat P70/2(RPM) -> Mux/2
  Right_Engine Jetcat P70/3(h (slg-ft^2/s)) -> Mux/3
  Right_Engine Jetcat P70/4(Fuel Pump Voltage (V)) -> Mux/4
  Right_Engine Jetcat P70/5(EGT (deg C)) -> Mux/5
  Right_Engine Jetcat P70/6(Fuel Flow (lbs/min)) -> Mux/6
  AC_Params2/1 -> Bus Selector5/1
  AC_Params1/1 -> Bus Selector3/1
  [THROTRC] -> Right_Engine Jetcat P70/1(Throttle)
  Bus Selector4/1 -> Left_Engine Jetcat P70/2(pratio)  "<pratio>"
  Bus Selector4/2 -> Left_Engine Jetcat P70/3(tratio)  "<tratio>"
  [Bypass] -> Left_Engine Jetcat P70/4(BypassDynamics)
  Bus Selector4/3 -> Left_Engine Jetcat P70/5(qbar)  "<qbar>"
  Bus Selector3/1 -> Left_Engine Jetcat P70/6(S)  "<S>"
  Bus Selector1/1 -> Right_Engine Jetcat P70/2(pratio)  "<pratio>"
  Bus Selector1/2 -> Right_Engine Jetcat P70/3(tratio)  "<tratio>"
  [Bypass] -> Right_Engine Jetcat P70/4(BypassDynamics)
  Bus Selector1/3 -> Right_Engine Jetcat P70/5(qbar)  "<qbar>"
  Bus Selector5/1 -> Right_Engine Jetcat P70/6(S)  "<S>"
  [THROTLC] -> Left_Engine Jetcat P70/1(Throttle)

== system gtm_design/GTM_T2/Gravity ==
  AuxVars : Inport
  Params : Inport  Port=2
  Bus Selector1 : BusSelector  OutputSignals=DCM
  Bus Selector6 : BusSelector  OutputSignals=mass
  Ground : Ground
  Ground1 : Ground
  Mux : Mux  Inputs=[3 3]
  Mux1 : Mux  Inputs=3
  Product : Product  Multiplication=Matrix(*)  RndMeth=Zero
  Product1 : Product  RndMeth=Zero
  acc due to gravity (ft/s^2) : Constant  Value=32.17405
  FM : Outport
  wires:
  acc due to gravity (ft/s^2)/1 -> Product1/2
  Ground1/1 -> Mux/2
  Product1/1 -> Mux1/3
  Ground/1 -> Mux1/2, Mux1/1
  Mux1/1 -> Product/2
  Mux/1 -> FM/1
  Product/1 -> Mux/1
  Params/1 -> Bus Selector6/1
  AuxVars/1 -> Bus Selector1/1
  Bus Selector1/1 -> Product/1  "<DCM>"
  Bus Selector6/1 -> Product1/1  "<mass>"
